simulink model "sf_custom_code_strings"  (R2025b)
settings: Solver=VariableStepAuto  StartTime=0.0  StopTime=10.0  RelTol=1e-3
settings Model: Creator=The MathWorks, Inc.  LastModifiedBy=The MathWorks, Inc.
settings SolverCC: AlgebraicLoopSolver=TrustRegion  DecoupledContinuousIntegration=on  MinimalZcImpactIntegration=on
settings DataIOCC: ReturnWorkspaceOutputs=off
settings OptimizationCC: ReuseModelBlockBuffer=off
settings DebuggingCC: StringTruncationChecking=none  UnconnectedInputMsg=warning  UnconnectedOutputMsg=warning  UnconnectedLineMsg=warning  ArithmeticOperatorsInVariantConditions=warning
settings ModelReferenceCC: EnableRefExpFcnMdlSchedulingChecks=on
settings SFSimCC: SimCustomHeaderCode="#include \"sf_custom_code_strings_functions.h\""  SimUserSources=sf_custom_code_strings_functions.c  SimUserIncludeDirs=.  SimUseLocalCustomCode=off
settings RTWCC: RTWUseLocalCustomCode=off  GPUComputeCapability=3.5

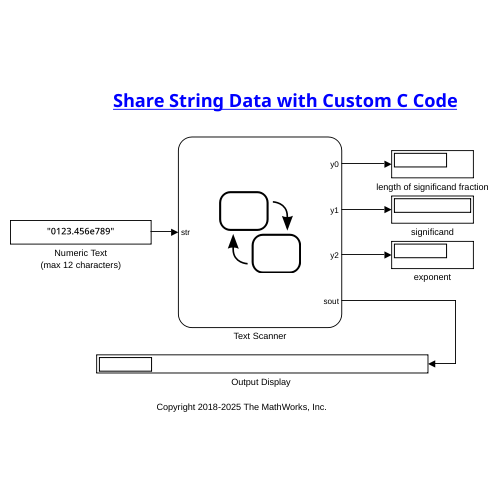
[thumbnail: Simulink's stored preview of the top-level diagram]
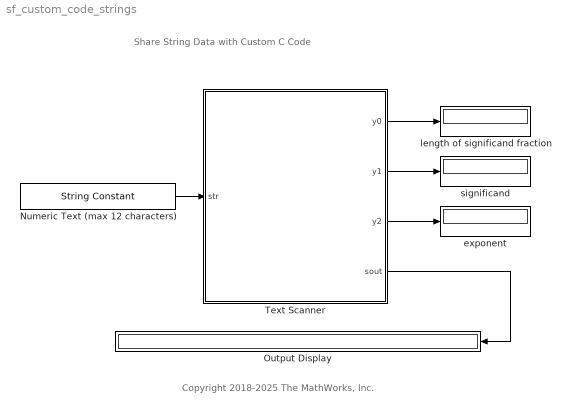
== system sf_custom_code_strings ==
  note: Copyright 2018-2025 The MathWorks, Inc.
  note: Share String Data with Custom C Code
  Numeric Text (max 12 characters) : StringConstant  String="\"0123.456e789\""  OutDataTypeStr=stringtype(12)
  "Output Display " : Display
  Text Scanner : Stateflow chart  TreatAsAtomicUnit=on
  exponent : Display
  length of significand fraction : Display
  significand : Display
  wires:
  Numeric Text (max 12 characters)/1 -> Text Scanner/1(str)
  Text Scanner/3(y2) -> exponent/1
  Text Scanner/2(y1) -> significand/1
  Text Scanner/4(sout) -> "Output Display "/1
  Text Scanner/1(y0) -> length of significand fraction/1

== stateflow chart sf_custom_code_strings/Text Scanner ==
  state Search
    entry:
    Astr = str2ascii(str,12);
    searchfun(n,Astr);
    % n[0] = number of leading zeroes
    % n[1] = characters before decimal point
    % n[2] = characters in significand
    % n[3] = length of string
  state Parse
    entry:
    y0 = n[2]-n[0]+(n[1]==n[2])-2;
    y1 = str2double(strcat("0",substr(str,0,n[2])))*pow(10,n[0]-n[1]+1);
    y2 = str2double(strcat("0",substr(str,n[2]+1,n[3]-n[2]-1)))+(n[1]-n[0]-1);
    % y0 = length of significand fraction
    % y1 = significand part of input
    % y2 = exponent part of input.
  state Merge
    entry:
    mergefun(Asout,Astr,y0,y1,y2);
    sout = ascii2str(Asout);
  (default) -> Search
  Search -> Parse
  Parse -> Merge
  data: y0 output int32; y1 output double; y2 output double; sout output string; Astr local uint8 size=[12]; Asout local uint8 size=[58]; str input; n local int32 size=4
